simulink model "acc_mpc"  (R2021b)
settings: Solver=ode5  StartTime=0.0  StopTime=80  FixedStep=1/20  RelTol=1e-3
PreLoadFcn:
  | mbxruntime.callbacks.PreLoadFcn(bdroot);
PostLoadFcn:
  | mbxruntime.callbacks.PostLoadFcn(bdroot);
InitFcn:
  | mbxruntime.callbacks.InitFcn(bdroot);
StartFcn:
  | mbxruntime.callbacks.StartFcn(bdroot);
StopFcn:
  | mbxruntime.callbacks.StopFcn(bdroot);
model workspace: external: MAT-File .\kea_demo_0218_cs_hws.mat (data not in the file)
undefined symbols (not defined in the file): DiscIntNeverNeededParam, kea_demo_0218_cs_1d5c9b61e8e009e5, kea_demo_0218_cs_4669f259e7287783, kea_demo_0218_cs_87ee11d7829c0052, kea_demo_0218_cs_Audi_A3_1_Dynamics_Simple_initialPitch, kea_demo_0218_cs_Audi_A3_1_Dynamics_Simple_initialRoll, kea_demo_0218_cs_Audi_A3_1_Dynamics_Simple_initialX, kea_demo_0218_cs_Audi_A3_1_Dynamics_Simple_initialY, kea_demo_0218_cs_Audi_A3_1_Dynamics_Simple_initialYaw, kea_demo_0218_cs_Audi_A3_1_Dynamics_Simple_initialZ, kea_demo_0218_cs_Audi_A3_1_PathFollower_Preview_1_PathUniqueID, kea_demo_0218_cs_Roewe_550_S_Sedan_1_Dynamics_Simple_initialX, kea_demo_0218_cs_Roewe_550_S_Sedan_1_Dynamics_Simple_initialY, kea_demo_0218_cs_Roewe_550_S_Sedan_1_Dynamics_Simple_initialYaw, kea_demo_0218_cs_Roewe_550_S_Sedan_1_Dynamics_Simple_initialZ, mbxruntime, warningInitialVelocity, x0
libraries: simulink x56, simulink_extras x18, mpcadaslib x1
(part 2 of 8)

== system acc_mpc/Synchronizer ==
  Bus Selector1 : BusSelector  OutputSignals=FederateStopped
  Stop Simulation : Stop
  sfun_Synchronizer : S-Function  FunctionName=sfun_Synchronizer  Parameters=SampleTime  SFunctionDeploymentMode=off  EnableBusSupport=off  mask(Legacy Function){SFunctionSpec=void prescan_synchronizer_outputFcn(void ** work1, PRESCAN_SYNCHRONIZEDATA y1[1]), SampleTime=TimeStep, ShowSpec=on}
      mask prompts: SampleTime "Sample time (-1 for inherited):"; ShowSpec "Display function specification"
      mask help:
      | This block allows you to call the legacy functions specified by the following Legacy Code Tool definition:
      | def.SFunctionName = 'sfun_Synchronizer';
      | def.OutputFcnSpec = 'void prescan_synchronizer_outputFcn(void ** work1, PRESCAN_TIMESTAMPDATA u1[1], PRESCAN_SYNCHRONIZEDATA y1[1])';
      | def.StartFcnSpec = 'void prescan_synchronizer_startFcn(void ** work1)';
      | def.TerminateFcnSpec = 'void prescan_synchronizer_terminateFcn(void ** work1)';
      | def.HeaderFiles = {'prescan_synchronizer_data.h'};
      | def.HostLibFiles = {'sensorinterfaced.lib'};
      | def.IncPaths = {'src', 'C:\prescandev\vislibrary\vis\..\pimp\include\sensors\InterfaceRTW'};
      | def.SrcPaths = {'src'};
      | def.LibPaths = {'C:\\prescandev\\vislibrary_build\lib'};
      | def.SampleTime = 'parameterized';
      | def.Options.language = 'C';
      mask Help: <p>This block was generated automatically by the Legacy Code Tool. For detailed help on this tool, call<a href="matlab:legacy_code('help')"> legacy_code('help')</a>.</p>
      mask Callback ShowSpec:
      | if strcmp(get_param(gcbh, 'ShowSpec'), 'on')
      |   set_param(gcbh, 'MaskDisplay', sprintf('fprintf(''%s'');', get_param(gcbh, 'SFunctionSpec')));
      | else
      |   set_param(gcbh, 'MaskDisplay', sprintf('fprintf(''%s'');', get_param(gcbh, 'FunctionName')));
      | end
      mask Display: fprintf('void prescan_synchronizer_outputFcn(void ** work1, PRESCAN_SYNCHRONIZEDATA y1[1])');
  wires:
  sfun_Synchronizer/1 -> Bus Selector1/1
  Bus Selector1/1 -> Stop Simulation/1  "<FederateStopped>"

== system acc_mpc/Audi_A3_1/AIR_1_Demux ==
  AIR : Inport  OutDataTypeStr=Bus: PRESCAN_AIRSENSORMESSAGE
  Activate_Switch : Subsystem
      mask Display: text(5,10,'')
  Bus Selector : BusSelector  OutputSignals=DATA.Range,DATA.Azimuth,DATA.Elevation,DATA.ID,DATA.Velocity,DATA.Heading,HEADER.timestamp
  Data Type Conversion : DataTypeConversion  OutDataTypeStr=double
  For Iterator : ForIterator  ResetStates=reset  IterationLimit=detectableObjects
  Selector : Selector  InputPortWidth=detectableObjects  IndexOptions=Index vector (port)  Indices=[1 3]  OutputSizes=1
  Signal2ArrayOfSignals1 : Subsystem  mask{VECTORLENGTH=detectableObjects}
      mask prompts: VECTORLENGTH "Length of vector"
  Signal2ArrayOfSignals2 : Subsystem  mask{VECTORLENGTH=detectableObjects}
      mask prompts: VECTORLENGTH "Length of vector"
  Signal2ArrayOfSignals3 : Subsystem  mask{VECTORLENGTH=detectableObjects}
      mask prompts: VECTORLENGTH "Length of vector"
  Signal2ArrayOfSignals4 : Subsystem  mask{VECTORLENGTH=detectableObjects}
      mask prompts: VECTORLENGTH "Length of vector"
  Signal2ArrayOfSignals5 : Subsystem  mask{VECTORLENGTH=detectableObjects}
      mask prompts: VECTORLENGTH "Length of vector"
  Signal2ArrayOfSignals6 : Subsystem  mask{VECTORLENGTH=detectableObjects}
      mask prompts: VECTORLENGTH "Length of vector"
  Signal2ArrayOfSignals7 : Subsystem  mask{VECTORLENGTH=detectableObjects}
      mask prompts: VECTORLENGTH "Length of vector"
  Range [m] : Outport  VectorParamsAs1DForOutWhenUnconnected=off
  Azimuth [deg] : Outport  Port=2  VectorParamsAs1DForOutWhenUnconnected=off
  Elevation [deg] : Outport  Port=3  VectorParamsAs1DForOutWhenUnconnected=off
  ID [-] : Outport  Port=4  VectorParamsAs1DForOutWhenUnconnected=off
  Velocity [m/s] : Outport  Port=5  VectorParamsAs1DForOutWhenUnconnected=off
  Heading [deg] : Outport  Port=6  VectorParamsAs1DForOutWhenUnconnected=off
  Timestamp [s] : Outport  Port=7  VectorParamsAs1DForOutWhenUnconnected=off
  wires:
  Signal2ArrayOfSignals7/1(ArrayofElements) -> Timestamp [s]/1
  Bus Selector/7 -> Signal2ArrayOfSignals7/2(Element)  "<timestamp>"
  Activate_Switch/1(On/Off) -> Heading [deg]/1
  AIR/1 -> Selector/1
  For Iterator/1 -> Signal2ArrayOfSignals6/1(LoopIndex), Signal2ArrayOfSignals5/1(LoopIndex), Signal2ArrayOfSignals4/1(LoopIndex), Signal2ArrayOfSignals3/1(LoopIndex), Signal2ArrayOfSignals1/1(LoopIndex), Signal2ArrayOfSignals2/1(LoopIndex), Signal2ArrayOfSignals7/1(LoopIndex), Selector/2
  Selector/1 -> Bus Selector/1
  Bus Selector/1 -> Signal2ArrayOfSignals2/2(Element)  "<Range>"
  Signal2ArrayOfSignals2/1(ArrayofElements) -> Range [m]/1
  Signal2ArrayOfSignals1/1(ArrayofElements) -> Azimuth [deg]/1
  Bus Selector/2 -> Signal2ArrayOfSignals1/2(Element)  "<Azimuth>"
  Signal2ArrayOfSignals3/1(ArrayofElements) -> Elevation [deg]/1
  Bus Selector/3 -> Signal2ArrayOfSignals3/2(Element)  "<Elevation>"
  Signal2ArrayOfSignals4/1(ArrayofElements) -> Activate_Switch/1(BeamID), Data Type Conversion/1
  Bus Selector/4 -> Signal2ArrayOfSignals4/2(Element)  "<ID>"
  Signal2ArrayOfSignals5/1(ArrayofElements) -> Velocity [m/s]/1
  Bus Selector/5 -> Signal2ArrayOfSignals5/2(Element)  "<Velocity>"
  Signal2ArrayOfSignals6/1(ArrayofElements) -> Activate_Switch/2(Heading)
  Bus Selector/6 -> Signal2ArrayOfSignals6/2(Element)  "<Heading>"
  Data Type Conversion/1 -> ID [-]/1

== system acc_mpc/Audi_A3_1/AIR_3_Demux ==
  AIR : Inport  OutDataTypeStr=Bus: PRESCAN_AIRSENSORMESSAGE
  Activate_Switch : Subsystem
      mask Display: text(5,10,'')
  Bus Selector : BusSelector  OutputSignals=DATA.Range,DATA.Azimuth,DATA.Elevation,DATA.ID,DATA.Velocity,DATA.Heading,HEADER.timestamp
  Data Type Conversion : DataTypeConversion  OutDataTypeStr=double
  For Iterator : ForIterator  ResetStates=reset  IterationLimit=detectableObjects
  Selector : Selector  InputPortWidth=detectableObjects  IndexOptions=Index vector (port)  Indices=[1 3]  OutputSizes=1
  Signal2ArrayOfSignals1 : Subsystem  mask{VECTORLENGTH=detectableObjects}
      mask prompts: VECTORLENGTH "Length of vector"
  Signal2ArrayOfSignals2 : Subsystem  mask{VECTORLENGTH=detectableObjects}
      mask prompts: VECTORLENGTH "Length of vector"
  Signal2ArrayOfSignals3 : Subsystem  mask{VECTORLENGTH=detectableObjects}
      mask prompts: VECTORLENGTH "Length of vector"
  Signal2ArrayOfSignals4 : Subsystem  mask{VECTORLENGTH=detectableObjects}
      mask prompts: VECTORLENGTH "Length of vector"
  Signal2ArrayOfSignals5 : Subsystem  mask{VECTORLENGTH=detectableObjects}
      mask prompts: VECTORLENGTH "Length of vector"
  Signal2ArrayOfSignals6 : Subsystem  mask{VECTORLENGTH=detectableObjects}
      mask prompts: VECTORLENGTH "Length of vector"
  Signal2ArrayOfSignals7 : Subsystem  mask{VECTORLENGTH=detectableObjects}
      mask prompts: VECTORLENGTH "Length of vector"
  Range [m] : Outport  VectorParamsAs1DForOutWhenUnconnected=off
  Azimuth [deg] : Outport  Port=2  VectorParamsAs1DForOutWhenUnconnected=off
  Elevation [deg] : Outport  Port=3  VectorParamsAs1DForOutWhenUnconnected=off
  ID [-] : Outport  Port=4  VectorParamsAs1DForOutWhenUnconnected=off
  Velocity [m/s] : Outport  Port=5  VectorParamsAs1DForOutWhenUnconnected=off
  Heading [deg] : Outport  Port=6  VectorParamsAs1DForOutWhenUnconnected=off
  Timestamp [s] : Outport  Port=7  VectorParamsAs1DForOutWhenUnconnected=off
  wires:
  Signal2ArrayOfSignals7/1(ArrayofElements) -> Timestamp [s]/1
  Bus Selector/7 -> Signal2ArrayOfSignals7/2(Element)  "<timestamp>"
  Activate_Switch/1(On/Off) -> Heading [deg]/1
  AIR/1 -> Selector/1
  For Iterator/1 -> Signal2ArrayOfSignals6/1(LoopIndex), Signal2ArrayOfSignals5/1(LoopIndex), Signal2ArrayOfSignals4/1(LoopIndex), Signal2ArrayOfSignals3/1(LoopIndex), Signal2ArrayOfSignals1/1(LoopIndex), Signal2ArrayOfSignals2/1(LoopIndex), Signal2ArrayOfSignals7/1(LoopIndex), Selector/2
  Selector/1 -> Bus Selector/1
  Bus Selector/1 -> Signal2ArrayOfSignals2/2(Element)  "<Range>"
  Signal2ArrayOfSignals2/1(ArrayofElements) -> Range [m]/1
  Signal2ArrayOfSignals1/1(ArrayofElements) -> Azimuth [deg]/1
  Bus Selector/2 -> Signal2ArrayOfSignals1/2(Element)  "<Azimuth>"
  Signal2ArrayOfSignals3/1(ArrayofElements) -> Elevation [deg]/1
  Bus Selector/3 -> Signal2ArrayOfSignals3/2(Element)  "<Elevation>"
  Signal2ArrayOfSignals4/1(ArrayofElements) -> Activate_Switch/1(BeamID), Data Type Conversion/1
  Bus Selector/4 -> Signal2ArrayOfSignals4/2(Element)  "<ID>"
  Signal2ArrayOfSignals5/1(ArrayofElements) -> Velocity [m/s]/1
  Bus Selector/5 -> Signal2ArrayOfSignals5/2(Element)  "<Velocity>"
  Signal2ArrayOfSignals6/1(ArrayofElements) -> Activate_Switch/2(Heading)
  Bus Selector/6 -> Signal2ArrayOfSignals6/2(Element)  "<Heading>"
  Data Type Conversion/1 -> ID [-]/1

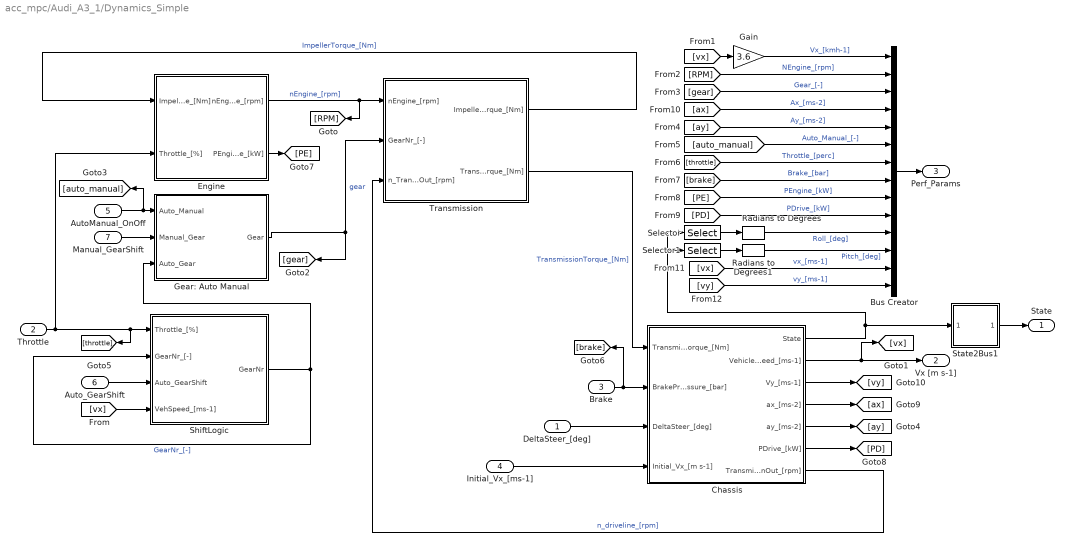
== system acc_mpc/Audi_A3_1/Dynamics_Simple ==
  DeltaSteer_[deg] : Inport
  Throttle : Inport  Port=2
  Brake : Inport  Port=3
  Initial_Vx_[ms-1] : Inport  Port=4
  AutoManual_OnOff : Inport  Port=5
  Auto_GearShift : Inport  Port=6
  Manual_GearShift : Inport  Port=7
  Bus Creator : BusCreator  Inputs=14
  Chassis : Subsystem
      mask Display: image(imread('Chassis.png'));
  Engine : Subsystem
      mask Display: image(imread('Engine.png'));
  Gain : Gain  Gain=3.6
  Gear: Auto Manual : Subsystem
  Radians to Degrees : simulink_extras/Transformations/Radians to Degrees
  Radians to Degrees1 : simulink_extras/Transformations/Radians to Degrees
  Selector : Selector  InputPortWidth=9  IndexOptions=Index vector (dialog)  Indices=7  OutputSizes=1
  Selector1 : Selector  InputPortWidth=9  IndexOptions=Index vector (dialog)  Indices=8  OutputSizes=1
  ShiftLogic : Subsystem
      mask Display: image(imread('Gearshift.png'));
  State2Bus1 : Subsystem  Tag=State  Priority=0  LoadFcn=load PrescanStateActuatorData  mask(PreScan Sink Block: State){x0=initialX, y0=initialY, z0=initialZ, Roll0=initialRoll, Pitch0=initialPitch, Yaw0=initialYaw, TimeStep=TimeStep}
      mask prompts: x0 "Ini x-position VEHICLE wrt GLOBAL axis system [m]"; y0 "Ini y-position VEHICLE wrt GLOBAL axis system [m]"; z0 "Ini z-position VEHICLE wrt GLOBAL axis system [m]"; Roll0 "Ini roll-angle BODY wrt VEHICLE axis system [deg]"; Pitch0 "Ini pitch-angle BODY wrt VEHICLE axis system [deg]"; Yaw0 "Ini yaw-angle VEHICLE wrt GLOBAL axis system [deg]"; TimeStep "Auto-Assigned: Upload Period [s]"
      mask help:
      | The Actor State contains a vector signal of size (9x1), containing the following signals:
      |
      | -  Position                  (x,y,z)                                     [m]
      | -  Velocity                  (vx,vy,vz)                               [m/s]
      | -  Angles                    (Roll, Pitch, Yaw)                   [rad]
      |
      | The Actor state is defined in the global axis system.
      | The state is superponed on the Initial position defined in the GUI.
      |
      | For more information, please click Help.
      settings: DeleteFcn=PreScanBlockDeleteFcn;
      mask Help: eval('openHelp(222)')
      mask Display: image(imread('State.png'))
  Transmission : Subsystem
      mask Display: image(imread('Transmission.png'));
  State : Outport  VectorParamsAs1DForOutWhenUnconnected=off
  Vx [m s-1] : Outport  Port=2  VectorParamsAs1DForOutWhenUnconnected=off
  Perf_Params : Outport  Port=3  VectorParamsAs1DForOutWhenUnconnected=off
  wires:
  State2Bus1/1(StateBus) -> State/1
  [vy] -> Bus Creator/14  "vy_[ms-1]"
  [vx] -> Bus Creator/13  "vx_[ms-1]"
  Chassis/7(TransmissionOut_[rpm]) -> Transmission/3(n_TransmissionOut_[rpm])  "n_driveline_[rpm]"
  Chassis/6(PDrive_[kW]) -> [PD]
  Chassis/5(ay_[ms-2]) -> [ay]
  Chassis/4(ax_[ms-2]) -> [ax]
  Chassis/3(Vy_[ms-1]) -> [vy]
  [vx] -> ShiftLogic/4(VehSpeed_[ms-1])
  Gear: Auto Manual/1(Gear) -> Transmission/2(GearNr_[-]), [gear]  "gear"
  Manual_GearShift/1 -> Gear: Auto Manual/2(Manual_Gear)
  AutoManual_OnOff/1 -> Gear: Auto Manual/1(Auto_Manual), [auto_manual]
  Chassis/2(VehicleSpeed_[ms-1]) -> [vx], Vx [m s-1]/1
  Auto_GearShift/1 -> ShiftLogic/3(Auto_GearShift)
  Throttle/1 -> Engine/2(Throttle_[%]), ShiftLogic/1(Throttle_[%]), [throttle]
  Initial_Vx_[ms-1]/1 -> Chassis/4(Initial_Vx_[m s-1])
  DeltaSteer_[deg]/1 -> Chassis/3(DeltaSteer_[deg])
  Chassis/1(State) -> Selector/1, Selector1/1, State2Bus1/1(State)
  Brake/1 -> [brake], Chassis/2(BrakePressure_[bar])
  Engine/1(nEngine_[rpm]) -> [RPM], Transmission/1(nEngine_[rpm])  "nEngine_[rpm]"
  ShiftLogic/1(GearNr) -> Gear: Auto Manual/3(Auto_Gear), ShiftLogic/2(GearNr_[-])  "GearNr_[-]"
  Transmission/2(TransmissionTorque_[Nm]) -> Chassis/1(TransmissionTorque_[Nm])  "TransmissionTorque_[Nm]"
  Transmission/1(ImpellerTorque_[Nm]) -> Engine/1(ImpellerTorque_[Nm])  "ImpellerTorque_[Nm]"
  Gain/1 -> Bus Creator/1  "Vx_[kmh-1]"
  [RPM] -> Bus Creator/2  "NEngine_[rpm]"
  [gear] -> Bus Creator/3  "Gear_[-]"
  [ay] -> Bus Creator/5  "Ay_[ms-2]"
  [auto_manual] -> Bus Creator/6  "Auto_Manual_[-]"
  [throttle] -> Bus Creator/7  "Throttle_[perc]"
  [brake] -> Bus Creator/8  "Brake_[bar]"
  Engine/2(PEngine_[kW]) -> [PE]
  Bus Creator/1 -> Perf_Params/1
  [PE] -> Bus Creator/9  "PEngine_[kW]"
  Radians to Degrees/1 -> Bus Creator/11  "Roll_[deg]"
  Radians to Degrees1/1 -> Bus Creator/12  "Pitch_[deg]"
  [PD] -> Bus Creator/10  "PDrive_[kW]"
  Selector/1 -> Radians to Degrees/1
  Selector1/1 -> Radians to Degrees1/1
  [vx] -> Gain/1
  [ax] -> Bus Creator/4  "Ax_[ms-2]"

== system acc_mpc/Audi_A3_1/PathFollower_Preview_1 ==
  ActorOffset_Left(+) / Right(-) [m] : Inport
  position x,y,Y [m,m,deg] : Inport  Port=2
  Initial Velocity [m/s] : Inport  Port=3
  Desired Velocity [m/s] : Inport  Port=4
  velocity [m/s] : Inport  Port=5
  vx [m/s] : Inport  Port=6
  vy [m/s] : Inport  Port=7
  Yaw rate [deg/s] : Inport  Port=8
  CorneringStiffness_Tyres_Front [N/rad] : Inport  Port=9
  CorneringStiffness_Tyres_Rear [N/rad] : Inport  Port=10
  steering_ratio[-] : Inport  Port=11
  LateralController : Subsystem
  LongitudinalController : Subsystem
  delta_steerwheel [deg] : Outport  VectorParamsAs1DForOutWhenUnconnected=off
  throttle [%] : Outport  Port=2  VectorParamsAs1DForOutWhenUnconnected=off
  brake pressure [bar] : Outport  Port=3  VectorParamsAs1DForOutWhenUnconnected=off
  v0 [m/s] : Outport  Port=4  VectorParamsAs1DForOutWhenUnconnected=off
  Auto_GearShift : Outport  Port=5  VectorParamsAs1DForOutWhenUnconnected=off
  Actor/Traj_distance [m] : Outport  Port=6  VectorParamsAs1DForOutWhenUnconnected=off
  Actor/Traj_angle [deg] : Outport  Port=7  VectorParamsAs1DForOutWhenUnconnected=off
  wires:
  LateralController/3(delta_steerwheel [deg]) -> delta_steerwheel [deg]/1
  steering_ratio[-]/1 -> LateralController/8(steering_ratio[-])
  CorneringStiffness_Tyres_Rear [N/rad]/1 -> LateralController/7(CorneringStiffness_Tyres_Rear [N/rad])
  CorneringStiffness_Tyres_Front [N/rad]/1 -> LateralController/6(CorneringStiffness_Tyres_Front [N/rad])
  Yaw rate [deg/s]/1 -> LateralController/5(Yaw rate [deg/s])
  vy [m/s]/1 -> LateralController/4(vy [m/s])
  vx [m/s]/1 -> LateralController/3(vx [m/s])
  position x,y,Y [m,m,deg]/1 -> LateralController/2(position x,y,Y [m,m,deg])
  ActorOffset_Left(+) / Right(-) [m]/1 -> LateralController/1(ActorOffset_Left(+) / Right(-) [m])
  LateralController/2(Actor/Traj_angle [deg]) -> Actor/Traj_angle [deg]/1
  LateralController/1(Actor/Traj_distance [m]) -> Actor/Traj_distance [m]/1
  velocity [m/s]/1 -> LongitudinalController/1(v_actual [m/s])
  LongitudinalController/1(throttle [%]) -> throttle [%]/1
  Desired Velocity [m/s]/1 -> LongitudinalController/2(Desired Velocity [m/s])
  Initial Velocity [m/s]/1 -> LongitudinalController/3(Initial Velocity [m/s])
  LongitudinalController/2(brake pressure [bar]) -> brake pressure [bar]/1
  LongitudinalController/3(v0 [m/s]) -> v0 [m/s]/1
  LongitudinalController/4(Auto_GearShift) -> Auto_GearShift/1

== system acc_mpc/Audi_A3_1/SELF_Demux ==
  SELF : Inport  OutDataTypeStr=Bus: PRESCAN_SELFSENSORDATA
  Bus Selector : BusSelector  OutputSignals=PositionX,PositionY,PositionZ,OrientationRoll,OrientationPitch,OrientationYaw,Velocity,Yaw_rate,Lat,Long,Alt,TimeStamp
  Demux2 : Demux  Outputs=3
  Gain : Gain  Gain=180/pi
  Gain1 : Gain  Gain=180/pi
  Vector Concatenate1 : Concatenate  NumInputs=3
  compas converter : Subsystem
  x [m] : Outport  VectorParamsAs1DForOutWhenUnconnected=off
  y [m] : Outport  Port=2  VectorParamsAs1DForOutWhenUnconnected=off
  z [m] : Outport  Port=3  VectorParamsAs1DForOutWhenUnconnected=off
  rotx [deg] : Outport  Port=4  VectorParamsAs1DForOutWhenUnconnected=off
  roty [deg] : Outport  Port=5  VectorParamsAs1DForOutWhenUnconnected=off
  rotz [deg] : Outport  Port=6  VectorParamsAs1DForOutWhenUnconnected=off
  GPS lat [deg] : Outport  Port=7  VectorParamsAs1DForOutWhenUnconnected=off
  GPS long [deg] : Outport  Port=8  VectorParamsAs1DForOutWhenUnconnected=off
  GPS alt [m] : Outport  Port=9  VectorParamsAs1DForOutWhenUnconnected=off
  velocity [m/s] : Outport  Port=10  VectorParamsAs1DForOutWhenUnconnected=off
  heading [deg] : Outport  Port=11  VectorParamsAs1DForOutWhenUnconnected=off
  yaw rate [deg/s] : Outport  Port=12  VectorParamsAs1DForOutWhenUnconnected=off
  TimeStamp [s] : Outport  Port=13  VectorParamsAs1DForOutWhenUnconnected=off
  wires:
  Bus Selector/12 -> TimeStamp [s]/1  "<TimeStamp>"
  Bus Selector/11 -> GPS alt [m]/1  "<Alt>"
  Bus Selector/10 -> GPS long [deg]/1  "<Long>"
  Bus Selector/9 -> GPS lat [deg]/1  "<Lat>"
  Bus Selector/8 -> Gain1/1  "<Yaw_rate>"
  Bus Selector/7 -> velocity [m/s]/1  "<Velocity>"
  Bus Selector/6 -> compas converter/1(rotz [rad]), Vector Concatenate1/3  "<OrientationYaw>"
  Bus Selector/5 -> Vector Concatenate1/2  "<OrientationPitch>"
  Bus Selector/4 -> Vector Concatenate1/1  "<OrientationRoll>"
  Vector Concatenate1/1 -> Gain/1
  Bus Selector/3 -> z [m]/1  "<PositionZ>"
  Bus Selector/2 -> y [m]/1  "<PositionY>"
  Bus Selector/1 -> x [m]/1  "<PositionX>"
  SELF/1 -> Bus Selector/1
  Gain/1 -> Demux2/1
  Demux2/1 -> rotx [deg]/1
  Demux2/2 -> roty [deg]/1
  Demux2/3 -> rotz [deg]/1
  compas converter/1(heading [deg]) -> heading [deg]/1
  Gain1/1 -> yaw rate [deg/s]/1

== system acc_mpc/Audi_A3_1/Speed ==
  BusSelector : BusSelector  OutputSignals=value
  sfun : S-Function  LoadFcn=load('PrescanScalarData.mat')  FunctionName=sfun_ProtobufScalarReader  Parameters=mbxruntime.parameters.convert(model), mbxruntime.parameters.convert(path), mbxruntime.parameters.convert(myType), mbxruntime.parameters.convert(timestep)  SFunctionDeploymentMode=off  EnableBusSupport=off  mask(PreScan Source Block: Protobuffer Scalar Reader){model=uint8(['pimp/scenariomodel' 0]), path=uint8(['catalogs/maneuverCatalog/maneuver:1/event:0/startConditions:0/condition:1/byEntity/speed/value' 0]), myType=uint8(['double' 0]), timestep=0}
      mask prompts: model "Data Model:"; path "Data Model Path:"; myType "Data Type:"; timestep "MATLAB timestep:"
      mask help:
      | This block reads a scalar value from the pb file.
      |
      | The supported data types are:
      | - double
      | - single
      | - uint32
      | - int32
      mask Display: fprintf('sfun')
  Speed : Outport
  wires:
  sfun/1 -> BusSelector/1
  BusSelector/1 -> Speed/1  "<value>"

== system acc_mpc/Audi_A3_1/State2PathFollowerCnv ==
  State BUS : Inport  OutDataTypeStr=Bus: PRESCAN_STATEACTUATORDATA
  Bus Selector : BusSelector  OutputSignals=AngularVelocityYaw,VelocityX,VelocityY,PositionX,PositionY,OrientationYaw
  Radians to Degrees : simulink_extras/Transformations/Radians to Degrees
  Radians to Degrees1 : simulink_extras/Transformations/Radians to Degrees
  SELF2PathFollowerMux : Mux  Tag=SELF2PathFollowerMux  Inputs=3
  velocity magnitude : Math  Operator=hypot  SignedPower=on  SaturateOnIntegerOverflow=on
  Yaw rate [deg/s] : Outport  VectorParamsAs1DForOutWhenUnconnected=off
  velocity [m/s] : Outport  Port=2  VectorParamsAs1DForOutWhenUnconnected=off
  position x,y,Y [m,m,deg] : Outport  Port=3  VectorParamsAs1DForOutWhenUnconnected=off
  wires:
  Radians to Degrees1/1 -> Yaw rate [deg/s]/1
  Bus Selector/1 -> Radians to Degrees1/1  "<AngularVelocityYaw>"
  velocity magnitude/1 -> velocity [m/s]/1
  SELF2PathFollowerMux/1 -> position x,y,Y [m,m,deg]/1
  State BUS/1 -> Bus Selector/1
  Bus Selector/2 -> velocity magnitude/1  "<VelocityX>"
  Bus Selector/3 -> velocity magnitude/2  "<VelocityY>"
  Radians to Degrees/1 -> SELF2PathFollowerMux/3
  Bus Selector/6 -> Radians to Degrees/1  "<OrientationYaw>"
  Bus Selector/4 -> SELF2PathFollowerMux/1  "<PositionX>"
  Bus Selector/5 -> SELF2PathFollowerMux/2  "<PositionY>"

== system acc_mpc/Audi_A3_1/Subsystem ==
  Acceleration : Inport
  Lead Val : Inport  Port=2
  If Action Subsystem : Subsystem  TreatAsAtomicUnit=on
  If Action Subsystem2 : Subsystem  TreatAsAtomicUnit=on
  If1 : If  IfExpression=u1==0
  Merge : Merge
  Merge1 : Merge
  Throttle : Outport
  Brake : Outport  Port=2
  wires:
  Lead Val/1 -> If1/1
  If1/2 -> If Action Subsystem2/Action
  Acceleration/1 -> If Action Subsystem2/1(Acceleration)
  If Action Subsystem2/1(Throttle) -> Merge/1
  If Action Subsystem2/2(Brake) -> Merge1/1
  Merge/1 -> Throttle/1
  If1/1 -> If Action Subsystem/Action
  If Action Subsystem/1(Throttle) -> Merge/2
  If Action Subsystem/2(Brake) -> Merge1/2
  Merge1/1 -> Brake/1

== system acc_mpc/Roewe_550_S_Sedan_1/AIR_2_Demux ==
  AIR : Inport  OutDataTypeStr=Bus: PRESCAN_AIRSENSORMESSAGE
  Activate_Switch : Subsystem
      mask Display: text(5,10,'')
  Bus Selector : BusSelector  OutputSignals=DATA.Range,DATA.Azimuth,DATA.Elevation,DATA.ID,DATA.Velocity,DATA.Heading,HEADER.timestamp
  Data Type Conversion : DataTypeConversion  OutDataTypeStr=double
  For Iterator : ForIterator  ResetStates=reset  IterationLimit=detectableObjects
  Selector : Selector  InputPortWidth=detectableObjects  IndexOptions=Index vector (port)  Indices=[1 3]  OutputSizes=1
  Signal2ArrayOfSignals1 : Subsystem  mask{VECTORLENGTH=detectableObjects}
      mask prompts: VECTORLENGTH "Length of vector"
  Signal2ArrayOfSignals2 : Subsystem  mask{VECTORLENGTH=detectableObjects}
      mask prompts: VECTORLENGTH "Length of vector"
  Signal2ArrayOfSignals3 : Subsystem  mask{VECTORLENGTH=detectableObjects}
      mask prompts: VECTORLENGTH "Length of vector"
  Signal2ArrayOfSignals4 : Subsystem  mask{VECTORLENGTH=detectableObjects}
      mask prompts: VECTORLENGTH "Length of vector"
  Signal2ArrayOfSignals5 : Subsystem  mask{VECTORLENGTH=detectableObjects}
      mask prompts: VECTORLENGTH "Length of vector"
  Signal2ArrayOfSignals6 : Subsystem  mask{VECTORLENGTH=detectableObjects}
      mask prompts: VECTORLENGTH "Length of vector"
  Signal2ArrayOfSignals7 : Subsystem  mask{VECTORLENGTH=detectableObjects}
      mask prompts: VECTORLENGTH "Length of vector"
  Range [m] : Outport  VectorParamsAs1DForOutWhenUnconnected=off
  Azimuth [deg] : Outport  Port=2  VectorParamsAs1DForOutWhenUnconnected=off
  Elevation [deg] : Outport  Port=3  VectorParamsAs1DForOutWhenUnconnected=off
  ID [-] : Outport  Port=4  VectorParamsAs1DForOutWhenUnconnected=off
  Velocity [m/s] : Outport  Port=5  VectorParamsAs1DForOutWhenUnconnected=off
  Heading [deg] : Outport  Port=6  VectorParamsAs1DForOutWhenUnconnected=off
  Timestamp [s] : Outport  Port=7  VectorParamsAs1DForOutWhenUnconnected=off
  wires:
  Signal2ArrayOfSignals7/1(ArrayofElements) -> Timestamp [s]/1
  Bus Selector/7 -> Signal2ArrayOfSignals7/2(Element)  "<timestamp>"
  Activate_Switch/1(On/Off) -> Heading [deg]/1
  AIR/1 -> Selector/1
  For Iterator/1 -> Signal2ArrayOfSignals6/1(LoopIndex), Signal2ArrayOfSignals5/1(LoopIndex), Signal2ArrayOfSignals4/1(LoopIndex), Signal2ArrayOfSignals3/1(LoopIndex), Signal2ArrayOfSignals1/1(LoopIndex), Signal2ArrayOfSignals2/1(LoopIndex), Signal2ArrayOfSignals7/1(LoopIndex), Selector/2
  Selector/1 -> Bus Selector/1
  Bus Selector/1 -> Signal2ArrayOfSignals2/2(Element)  "<Range>"
  Signal2ArrayOfSignals2/1(ArrayofElements) -> Range [m]/1
  Signal2ArrayOfSignals1/1(ArrayofElements) -> Azimuth [deg]/1
  Bus Selector/2 -> Signal2ArrayOfSignals1/2(Element)  "<Azimuth>"
  Signal2ArrayOfSignals3/1(ArrayofElements) -> Elevation [deg]/1
  Bus Selector/3 -> Signal2ArrayOfSignals3/2(Element)  "<Elevation>"
  Signal2ArrayOfSignals4/1(ArrayofElements) -> Activate_Switch/1(BeamID), Data Type Conversion/1
  Bus Selector/4 -> Signal2ArrayOfSignals4/2(Element)  "<ID>"
  Signal2ArrayOfSignals5/1(ArrayofElements) -> Velocity [m/s]/1
  Bus Selector/5 -> Signal2ArrayOfSignals5/2(Element)  "<Velocity>"
  Signal2ArrayOfSignals6/1(ArrayofElements) -> Activate_Switch/2(Heading)
  Bus Selector/6 -> Signal2ArrayOfSignals6/2(Element)  "<Heading>"
  Data Type Conversion/1 -> ID [-]/1

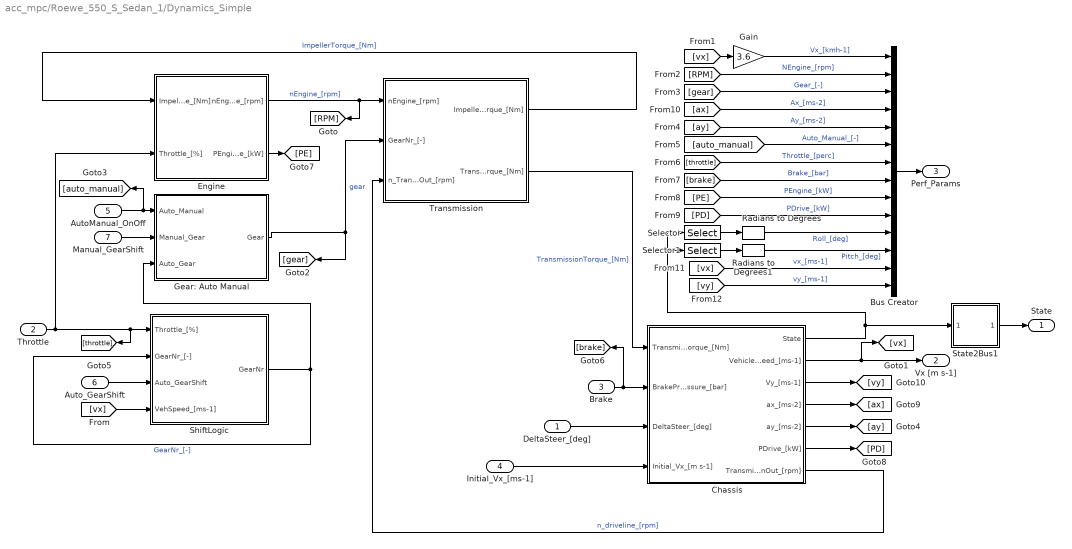
== system acc_mpc/Roewe_550_S_Sedan_1/Dynamics_Simple ==
  DeltaSteer_[deg] : Inport
  Throttle : Inport  Port=2
  Brake : Inport  Port=3
  Initial_Vx_[ms-1] : Inport  Port=4
  AutoManual_OnOff : Inport  Port=5
  Auto_GearShift : Inport  Port=6
  Manual_GearShift : Inport  Port=7
  Bus Creator : BusCreator  Inputs=14
  Chassis : Subsystem
      mask Display: image(imread('Chassis.png'));
  Engine : Subsystem
      mask Display: image(imread('Engine.png'));
  Gain : Gain  Gain=3.6
  Gear: Auto Manual : Subsystem
  Radians to Degrees : simulink_extras/Transformations/Radians to Degrees
  Radians to Degrees1 : simulink_extras/Transformations/Radians to Degrees
  Selector : Selector  InputPortWidth=9  IndexOptions=Index vector (dialog)  Indices=7  OutputSizes=1
  Selector1 : Selector  InputPortWidth=9  IndexOptions=Index vector (dialog)  Indices=8  OutputSizes=1
  ShiftLogic : Subsystem
      mask Display: image(imread('Gearshift.png'));
  State2Bus1 : Subsystem  Tag=State  Priority=0  LoadFcn=load PrescanStateActuatorData  mask(PreScan Sink Block: State){x0=initialX, y0=initialY, z0=initialZ, Roll0=initialRoll, Pitch0=initialPitch, Yaw0=initialYaw, TimeStep=TimeStep}
      mask prompts: x0 "Ini x-position VEHICLE wrt GLOBAL axis system [m]"; y0 "Ini y-position VEHICLE wrt GLOBAL axis system [m]"; z0 "Ini z-position VEHICLE wrt GLOBAL axis system [m]"; Roll0 "Ini roll-angle BODY wrt VEHICLE axis system [deg]"; Pitch0 "Ini pitch-angle BODY wrt VEHICLE axis system [deg]"; Yaw0 "Ini yaw-angle VEHICLE wrt GLOBAL axis system [deg]"; TimeStep "Auto-Assigned: Upload Period [s]"
      mask help:
      | The Actor State contains a vector signal of size (9x1), containing the following signals:
      |
      | -  Position                  (x,y,z)                                     [m]
      | -  Velocity                  (vx,vy,vz)                               [m/s]
      | -  Angles                    (Roll, Pitch, Yaw)                   [rad]
      |
      | The Actor state is defined in the global axis system.
      | The state is superponed on the Initial position defined in the GUI.
      |
      | For more information, please click Help.
      settings: DeleteFcn=PreScanBlockDeleteFcn;
      mask Help: eval('openHelp(222)')
      mask Display: image(imread('State.png'))
  Transmission : Subsystem
      mask Display: image(imread('Transmission.png'));
  State : Outport  VectorParamsAs1DForOutWhenUnconnected=off
  Vx [m s-1] : Outport  Port=2  VectorParamsAs1DForOutWhenUnconnected=off
  Perf_Params : Outport  Port=3  VectorParamsAs1DForOutWhenUnconnected=off
  wires:
  State2Bus1/1(StateBus) -> State/1
  [vy] -> Bus Creator/14  "vy_[ms-1]"
  [vx] -> Bus Creator/13  "vx_[ms-1]"
  Chassis/7(TransmissionOut_[rpm]) -> Transmission/3(n_TransmissionOut_[rpm])  "n_driveline_[rpm]"
  Chassis/6(PDrive_[kW]) -> [PD]
  Chassis/5(ay_[ms-2]) -> [ay]
  Chassis/4(ax_[ms-2]) -> [ax]
  Chassis/3(Vy_[ms-1]) -> [vy]
  [vx] -> ShiftLogic/4(VehSpeed_[ms-1])
  Gear: Auto Manual/1(Gear) -> Transmission/2(GearNr_[-]), [gear]  "gear"
  Manual_GearShift/1 -> Gear: Auto Manual/2(Manual_Gear)
  AutoManual_OnOff/1 -> Gear: Auto Manual/1(Auto_Manual), [auto_manual]
  Chassis/2(VehicleSpeed_[ms-1]) -> [vx], Vx [m s-1]/1
  Auto_GearShift/1 -> ShiftLogic/3(Auto_GearShift)
  Throttle/1 -> Engine/2(Throttle_[%]), ShiftLogic/1(Throttle_[%]), [throttle]
  Initial_Vx_[ms-1]/1 -> Chassis/4(Initial_Vx_[m s-1])
  DeltaSteer_[deg]/1 -> Chassis/3(DeltaSteer_[deg])
  Chassis/1(State) -> Selector/1, Selector1/1, State2Bus1/1(State)
  Brake/1 -> [brake], Chassis/2(BrakePressure_[bar])
  Engine/1(nEngine_[rpm]) -> [RPM], Transmission/1(nEngine_[rpm])  "nEngine_[rpm]"
  ShiftLogic/1(GearNr) -> Gear: Auto Manual/3(Auto_Gear), ShiftLogic/2(GearNr_[-])  "GearNr_[-]"
  Transmission/2(TransmissionTorque_[Nm]) -> Chassis/1(TransmissionTorque_[Nm])  "TransmissionTorque_[Nm]"
  Transmission/1(ImpellerTorque_[Nm]) -> Engine/1(ImpellerTorque_[Nm])  "ImpellerTorque_[Nm]"
  Gain/1 -> Bus Creator/1  "Vx_[kmh-1]"
  [RPM] -> Bus Creator/2  "NEngine_[rpm]"
  [gear] -> Bus Creator/3  "Gear_[-]"
  [ay] -> Bus Creator/5  "Ay_[ms-2]"
  [auto_manual] -> Bus Creator/6  "Auto_Manual_[-]"
  [throttle] -> Bus Creator/7  "Throttle_[perc]"
  [brake] -> Bus Creator/8  "Brake_[bar]"
  Engine/2(PEngine_[kW]) -> [PE]
  Bus Creator/1 -> Perf_Params/1
  [PE] -> Bus Creator/9  "PEngine_[kW]"
  Radians to Degrees/1 -> Bus Creator/11  "Roll_[deg]"
  Radians to Degrees1/1 -> Bus Creator/12  "Pitch_[deg]"
  [PD] -> Bus Creator/10  "PDrive_[kW]"
  Selector/1 -> Radians to Degrees/1
  Selector1/1 -> Radians to Degrees1/1
  [vx] -> Gain/1
  [ax] -> Bus Creator/4  "Ax_[ms-2]"

== system acc_mpc/Roewe_550_S_Sedan_1/PathFollower_Preview_1 ==
  ActorOffset_Left(+) / Right(-) [m] : Inport
  position x,y,Y [m,m,deg] : Inport  Port=2
  Initial Velocity [m/s] : Inport  Port=3
  Desired Velocity [m/s] : Inport  Port=4
  velocity [m/s] : Inport  Port=5
  vx [m/s] : Inport  Port=6
  vy [m/s] : Inport  Port=7
  Yaw rate [deg/s] : Inport  Port=8
  CorneringStiffness_Tyres_Front [N/rad] : Inport  Port=9
  CorneringStiffness_Tyres_Rear [N/rad] : Inport  Port=10
  steering_ratio[-] : Inport  Port=11
  LateralController : Subsystem
  LongitudinalController : Subsystem
  delta_steerwheel [deg] : Outport  VectorParamsAs1DForOutWhenUnconnected=off
  throttle [%] : Outport  Port=2  VectorParamsAs1DForOutWhenUnconnected=off
  brake pressure [bar] : Outport  Port=3  VectorParamsAs1DForOutWhenUnconnected=off
  v0 [m/s] : Outport  Port=4  VectorParamsAs1DForOutWhenUnconnected=off
  Auto_GearShift : Outport  Port=5  VectorParamsAs1DForOutWhenUnconnected=off
  Actor/Traj_distance [m] : Outport  Port=6  VectorParamsAs1DForOutWhenUnconnected=off
  Actor/Traj_angle [deg] : Outport  Port=7  VectorParamsAs1DForOutWhenUnconnected=off
  wires:
  LateralController/3(delta_steerwheel [deg]) -> delta_steerwheel [deg]/1
  steering_ratio[-]/1 -> LateralController/8(steering_ratio[-])
  CorneringStiffness_Tyres_Rear [N/rad]/1 -> LateralController/7(CorneringStiffness_Tyres_Rear [N/rad])
  CorneringStiffness_Tyres_Front [N/rad]/1 -> LateralController/6(CorneringStiffness_Tyres_Front [N/rad])
  Yaw rate [deg/s]/1 -> LateralController/5(Yaw rate [deg/s])
  vy [m/s]/1 -> LateralController/4(vy [m/s])
  vx [m/s]/1 -> LateralController/3(vx [m/s])
  position x,y,Y [m,m,deg]/1 -> LateralController/2(position x,y,Y [m,m,deg])
  ActorOffset_Left(+) / Right(-) [m]/1 -> LateralController/1(ActorOffset_Left(+) / Right(-) [m])
  LateralController/2(Actor/Traj_angle [deg]) -> Actor/Traj_angle [deg]/1
  LateralController/1(Actor/Traj_distance [m]) -> Actor/Traj_distance [m]/1
  velocity [m/s]/1 -> LongitudinalController/1(v_actual [m/s])
  LongitudinalController/1(throttle [%]) -> throttle [%]/1
  Desired Velocity [m/s]/1 -> LongitudinalController/2(Desired Velocity [m/s])
  Initial Velocity [m/s]/1 -> LongitudinalController/3(Initial Velocity [m/s])
  LongitudinalController/2(brake pressure [bar]) -> brake pressure [bar]/1
  LongitudinalController/3(v0 [m/s]) -> v0 [m/s]/1
  LongitudinalController/4(Auto_GearShift) -> Auto_GearShift/1

== system acc_mpc/Roewe_550_S_Sedan_1/SELF_Demux ==
  SELF : Inport  OutDataTypeStr=Bus: PRESCAN_SELFSENSORDATA
  Bus Selector : BusSelector  OutputSignals=PositionX,PositionY,PositionZ,OrientationRoll,OrientationPitch,OrientationYaw,Velocity,Yaw_rate,Lat,Long,Alt,TimeStamp
  Demux2 : Demux  Outputs=3
  Gain : Gain  Gain=180/pi
  Gain1 : Gain  Gain=180/pi
  Vector Concatenate1 : Concatenate  NumInputs=3
  compas converter : Subsystem
  x [m] : Outport  VectorParamsAs1DForOutWhenUnconnected=off
  y [m] : Outport  Port=2  VectorParamsAs1DForOutWhenUnconnected=off
  z [m] : Outport  Port=3  VectorParamsAs1DForOutWhenUnconnected=off
  rotx [deg] : Outport  Port=4  VectorParamsAs1DForOutWhenUnconnected=off
  roty [deg] : Outport  Port=5  VectorParamsAs1DForOutWhenUnconnected=off
  rotz [deg] : Outport  Port=6  VectorParamsAs1DForOutWhenUnconnected=off
  GPS lat [deg] : Outport  Port=7  VectorParamsAs1DForOutWhenUnconnected=off
  GPS long [deg] : Outport  Port=8  VectorParamsAs1DForOutWhenUnconnected=off
  GPS alt [m] : Outport  Port=9  VectorParamsAs1DForOutWhenUnconnected=off
  velocity [m/s] : Outport  Port=10  VectorParamsAs1DForOutWhenUnconnected=off
  heading [deg] : Outport  Port=11  VectorParamsAs1DForOutWhenUnconnected=off
  yaw rate [deg/s] : Outport  Port=12  VectorParamsAs1DForOutWhenUnconnected=off
  TimeStamp [s] : Outport  Port=13  VectorParamsAs1DForOutWhenUnconnected=off
  wires:
  Bus Selector/12 -> TimeStamp [s]/1  "<TimeStamp>"
  Bus Selector/11 -> GPS alt [m]/1  "<Alt>"
  Bus Selector/10 -> GPS long [deg]/1  "<Long>"
  Bus Selector/9 -> GPS lat [deg]/1  "<Lat>"
  Bus Selector/8 -> Gain1/1  "<Yaw_rate>"
  Bus Selector/7 -> velocity [m/s]/1  "<Velocity>"
  Bus Selector/6 -> compas converter/1(rotz [rad]), Vector Concatenate1/3  "<OrientationYaw>"
  Bus Selector/5 -> Vector Concatenate1/2  "<OrientationPitch>"
  Bus Selector/4 -> Vector Concatenate1/1  "<OrientationRoll>"
  Vector Concatenate1/1 -> Gain/1
  Bus Selector/3 -> z [m]/1  "<PositionZ>"
  Bus Selector/2 -> y [m]/1  "<PositionY>"
  Bus Selector/1 -> x [m]/1  "<PositionX>"
  SELF/1 -> Bus Selector/1
  Gain/1 -> Demux2/1
  Demux2/1 -> rotx [deg]/1
  Demux2/2 -> roty [deg]/1
  Demux2/3 -> rotz [deg]/1
  compas converter/1(heading [deg]) -> heading [deg]/1
  Gain1/1 -> yaw rate [deg/s]/1

== system acc_mpc/Roewe_550_S_Sedan_1/Speed ==
  BusSelector : BusSelector  OutputSignals=value
  sfun : S-Function  LoadFcn=load('PrescanScalarData.mat')  FunctionName=sfun_ProtobufScalarReader  Parameters=mbxruntime.parameters.convert(model), mbxruntime.parameters.convert(path), mbxruntime.parameters.convert(myType), mbxruntime.parameters.convert(timestep)  SFunctionDeploymentMode=off  EnableBusSupport=off  mask(PreScan Source Block: Protobuffer Scalar Reader){model=uint8(['pimp/scenariomodel' 0]), path=uint8(['catalogs/maneuverCatalog/maneuver:0/event:0/startConditions:0/condition:1/byEntity/speed/value' 0]), myType=uint8(['double' 0]), timestep=0}
      mask prompts: model "Data Model:"; path "Data Model Path:"; myType "Data Type:"; timestep "MATLAB timestep:"
      mask help:
      | This block reads a scalar value from the pb file.
      |
      | The supported data types are:
      | - double
      | - single
      | - uint32
      | - int32
      mask Display: fprintf('sfun')
  Speed : Outport
  wires:
  sfun/1 -> BusSelector/1
  BusSelector/1 -> Speed/1  "<value>"

== system acc_mpc/Roewe_550_S_Sedan_1/State2PathFollowerCnv ==
  State BUS : Inport  OutDataTypeStr=Bus: PRESCAN_STATEACTUATORDATA
  Bus Selector : BusSelector  OutputSignals=AngularVelocityYaw,VelocityX,VelocityY,PositionX,PositionY,OrientationYaw
  Radians to Degrees : simulink_extras/Transformations/Radians to Degrees
  Radians to Degrees1 : simulink_extras/Transformations/Radians to Degrees
  SELF2PathFollowerMux : Mux  Tag=SELF2PathFollowerMux  Inputs=3
  velocity magnitude : Math  Operator=hypot  SignedPower=on  SaturateOnIntegerOverflow=on
  Yaw rate [deg/s] : Outport  VectorParamsAs1DForOutWhenUnconnected=off
  velocity [m/s] : Outport  Port=2  VectorParamsAs1DForOutWhenUnconnected=off
  position x,y,Y [m,m,deg] : Outport  Port=3  VectorParamsAs1DForOutWhenUnconnected=off
  wires:
  Radians to Degrees1/1 -> Yaw rate [deg/s]/1
  Bus Selector/1 -> Radians to Degrees1/1  "<AngularVelocityYaw>"
  velocity magnitude/1 -> velocity [m/s]/1
  SELF2PathFollowerMux/1 -> position x,y,Y [m,m,deg]/1
  State BUS/1 -> Bus Selector/1
  Bus Selector/2 -> velocity magnitude/1  "<VelocityX>"
  Bus Selector/3 -> velocity magnitude/2  "<VelocityY>"
  Radians to Degrees/1 -> SELF2PathFollowerMux/3
  Bus Selector/6 -> Radians to Degrees/1  "<OrientationYaw>"
  Bus Selector/4 -> SELF2PathFollowerMux/1  "<PositionX>"
  Bus Selector/5 -> SELF2PathFollowerMux/2  "<PositionY>"

== system acc_mpc/Audi_A3_1/AIR_1_Demux/Activate_Switch ==
  BeamID : Inport
  Heading : Inport  Port=2
  Constant : Constant  Value=0
  Product1 : Product  RndMeth=Zero
  Relational Operator : RelationalOperator  Operator=~=  OutDataTypeStr=boolean  RndMeth=Nearest
  On/Off : Outport  VectorParamsAs1DForOutWhenUnconnected=off
  wires:
  Heading/1 -> Product1/2
  Product1/1 -> On/Off/1
  BeamID/1 -> Relational Operator/2
  Relational Operator/1 -> Product1/1
  Constant/1 -> Relational Operator/1

== system acc_mpc/Audi_A3_1/AIR_1_Demux/Signal2ArrayOfSignals1 ==
  note: Initial state of Previous vector block
      | set to zeros(VECTORLENGTH,1)
  note: Set mask parameter VECTORLENGTH
      |  to MAXMESSAGES
  LoopIndex : Inport
  Element : Inport  Port=2
  Assignment : Assignment  IndexOptions=Index vector (port)  Indices=1  OutputSizes=1
  Previous vector : Memory  InitialCondition=zeros(VECTORLENGTH,1)  InheritSampleTime=on
  ArrayofElements : Outport  VectorParamsAs1DForOutWhenUnconnected=off
  wires:
  Assignment/1 -> Previous vector/1, ArrayofElements/1
  Previous vector/1 -> Assignment/1
  LoopIndex/1 -> Assignment/3
  Element/1 -> Assignment/2

== system acc_mpc/Audi_A3_1/AIR_1_Demux/Signal2ArrayOfSignals2 ==
  note: Initial state of Previous vector block
      | set to zeros(VECTORLENGTH,1)
  note: Set mask parameter VECTORLENGTH
      |  to MAXMESSAGES
  LoopIndex : Inport
  Element : Inport  Port=2
  Assignment : Assignment  IndexOptions=Index vector (port)  Indices=1  OutputSizes=1
  Previous vector : Memory  InitialCondition=zeros(VECTORLENGTH,1)  InheritSampleTime=on
  ArrayofElements : Outport  VectorParamsAs1DForOutWhenUnconnected=off
  wires:
  Assignment/1 -> Previous vector/1, ArrayofElements/1
  Previous vector/1 -> Assignment/1
  LoopIndex/1 -> Assignment/3
  Element/1 -> Assignment/2

== system acc_mpc/Audi_A3_1/AIR_1_Demux/Signal2ArrayOfSignals3 ==
  note: Initial state of Previous vector block
      | set to zeros(VECTORLENGTH,1)
  note: Set mask parameter VECTORLENGTH
      |  to MAXMESSAGES
  LoopIndex : Inport
  Element : Inport  Port=2
  Assignment : Assignment  IndexOptions=Index vector (port)  Indices=1  OutputSizes=1
  Previous vector : Memory  InitialCondition=zeros(VECTORLENGTH,1)  InheritSampleTime=on
  ArrayofElements : Outport  VectorParamsAs1DForOutWhenUnconnected=off
  wires:
  Assignment/1 -> Previous vector/1, ArrayofElements/1
  Previous vector/1 -> Assignment/1
  LoopIndex/1 -> Assignment/3
  Element/1 -> Assignment/2

== system acc_mpc/Audi_A3_1/AIR_1_Demux/Signal2ArrayOfSignals4 ==
  note: Initial state of Previous vector block
      | set to zeros(VECTORLENGTH,1)
  note: Set mask parameter VECTORLENGTH
      |  to MAXMESSAGES
  LoopIndex : Inport
  Element : Inport  Port=2
  Assignment : Assignment  IndexOptions=Index vector (port)  Indices=1  OutputSizes=1
  Previous vector : Memory  InitialCondition=zeros(VECTORLENGTH,1)  InheritSampleTime=on
  ArrayofElements : Outport  VectorParamsAs1DForOutWhenUnconnected=off
  wires:
  Assignment/1 -> Previous vector/1, ArrayofElements/1
  Previous vector/1 -> Assignment/1
  LoopIndex/1 -> Assignment/3
  Element/1 -> Assignment/2

== system acc_mpc/Audi_A3_1/AIR_1_Demux/Signal2ArrayOfSignals5 ==
  note: Initial state of Previous vector block
      | set to zeros(VECTORLENGTH,1)
  note: Set mask parameter VECTORLENGTH
      |  to MAXMESSAGES
  LoopIndex : Inport
  Element : Inport  Port=2
  Assignment : Assignment  IndexOptions=Index vector (port)  Indices=1  OutputSizes=1
  Previous vector : Memory  InitialCondition=zeros(VECTORLENGTH,1)  InheritSampleTime=on
  ArrayofElements : Outport  VectorParamsAs1DForOutWhenUnconnected=off
  wires:
  Assignment/1 -> Previous vector/1, ArrayofElements/1
  Previous vector/1 -> Assignment/1
  LoopIndex/1 -> Assignment/3
  Element/1 -> Assignment/2

== system acc_mpc/Audi_A3_1/AIR_1_Demux/Signal2ArrayOfSignals6 ==
  note: Initial state of Previous vector block
      | set to zeros(VECTORLENGTH,1)
  note: Set mask parameter VECTORLENGTH
      |  to MAXMESSAGES
  LoopIndex : Inport
  Element : Inport  Port=2
  Assignment : Assignment  IndexOptions=Index vector (port)  Indices=1  OutputSizes=1
  Previous vector : Memory  InitialCondition=zeros(VECTORLENGTH,1)  InheritSampleTime=on
  ArrayofElements : Outport  VectorParamsAs1DForOutWhenUnconnected=off
  wires:
  Assignment/1 -> Previous vector/1, ArrayofElements/1
  Previous vector/1 -> Assignment/1
  LoopIndex/1 -> Assignment/3
  Element/1 -> Assignment/2

== system acc_mpc/Audi_A3_1/AIR_1_Demux/Signal2ArrayOfSignals7 ==
  note: Initial state of Previous vector block
      | set to zeros(VECTORLENGTH,1)
  note: Set mask parameter VECTORLENGTH
      |  to MAXMESSAGES
  LoopIndex : Inport
  Element : Inport  Port=2
  Assignment : Assignment  IndexOptions=Index vector (port)  Indices=1  OutputSizes=1
  Previous vector : Memory  InitialCondition=zeros(VECTORLENGTH,1)  InheritSampleTime=on
  ArrayofElements : Outport  VectorParamsAs1DForOutWhenUnconnected=off
  wires:
  Assignment/1 -> Previous vector/1, ArrayofElements/1
  Previous vector/1 -> Assignment/1
  LoopIndex/1 -> Assignment/3
  Element/1 -> Assignment/2

== system acc_mpc/Audi_A3_1/AIR_3_Demux/Activate_Switch ==
  BeamID : Inport
  Heading : Inport  Port=2
  Constant : Constant  Value=0
  Product1 : Product  RndMeth=Zero
  Relational Operator : RelationalOperator  Operator=~=  OutDataTypeStr=boolean  RndMeth=Nearest
  On/Off : Outport  VectorParamsAs1DForOutWhenUnconnected=off
  wires:
  Heading/1 -> Product1/2
  Product1/1 -> On/Off/1
  BeamID/1 -> Relational Operator/2
  Relational Operator/1 -> Product1/1
  Constant/1 -> Relational Operator/1

== system acc_mpc/Audi_A3_1/AIR_3_Demux/Signal2ArrayOfSignals1 ==
  note: Initial state of Previous vector block
      | set to zeros(VECTORLENGTH,1)
  note: Set mask parameter VECTORLENGTH
      |  to MAXMESSAGES
  LoopIndex : Inport
  Element : Inport  Port=2
  Assignment : Assignment  IndexOptions=Index vector (port)  Indices=1  OutputSizes=1
  Previous vector : Memory  InitialCondition=zeros(VECTORLENGTH,1)  InheritSampleTime=on
  ArrayofElements : Outport  VectorParamsAs1DForOutWhenUnconnected=off
  wires:
  Assignment/1 -> Previous vector/1, ArrayofElements/1
  Previous vector/1 -> Assignment/1
  LoopIndex/1 -> Assignment/3
  Element/1 -> Assignment/2

== system acc_mpc/Audi_A3_1/AIR_3_Demux/Signal2ArrayOfSignals2 ==
  note: Initial state of Previous vector block
      | set to zeros(VECTORLENGTH,1)
  note: Set mask parameter VECTORLENGTH
      |  to MAXMESSAGES
  LoopIndex : Inport
  Element : Inport  Port=2
  Assignment : Assignment  IndexOptions=Index vector (port)  Indices=1  OutputSizes=1
  Previous vector : Memory  InitialCondition=zeros(VECTORLENGTH,1)  InheritSampleTime=on
  ArrayofElements : Outport  VectorParamsAs1DForOutWhenUnconnected=off
  wires:
  Assignment/1 -> Previous vector/1, ArrayofElements/1
  Previous vector/1 -> Assignment/1
  LoopIndex/1 -> Assignment/3
  Element/1 -> Assignment/2

== system acc_mpc/Audi_A3_1/AIR_3_Demux/Signal2ArrayOfSignals3 ==
  note: Initial state of Previous vector block
      | set to zeros(VECTORLENGTH,1)
  note: Set mask parameter VECTORLENGTH
      |  to MAXMESSAGES
  LoopIndex : Inport
  Element : Inport  Port=2
  Assignment : Assignment  IndexOptions=Index vector (port)  Indices=1  OutputSizes=1
  Previous vector : Memory  InitialCondition=zeros(VECTORLENGTH,1)  InheritSampleTime=on
  ArrayofElements : Outport  VectorParamsAs1DForOutWhenUnconnected=off
  wires:
  Assignment/1 -> Previous vector/1, ArrayofElements/1
  Previous vector/1 -> Assignment/1
  LoopIndex/1 -> Assignment/3
  Element/1 -> Assignment/2

== system acc_mpc/Audi_A3_1/AIR_3_Demux/Signal2ArrayOfSignals4 ==
  note: Initial state of Previous vector block
      | set to zeros(VECTORLENGTH,1)
  note: Set mask parameter VECTORLENGTH
      |  to MAXMESSAGES
  LoopIndex : Inport
  Element : Inport  Port=2
  Assignment : Assignment  IndexOptions=Index vector (port)  Indices=1  OutputSizes=1
  Previous vector : Memory  InitialCondition=zeros(VECTORLENGTH,1)  InheritSampleTime=on
  ArrayofElements : Outport  VectorParamsAs1DForOutWhenUnconnected=off
  wires:
  Assignment/1 -> Previous vector/1, ArrayofElements/1
  Previous vector/1 -> Assignment/1
  LoopIndex/1 -> Assignment/3
  Element/1 -> Assignment/2

== system acc_mpc/Audi_A3_1/AIR_3_Demux/Signal2ArrayOfSignals5 ==
  note: Initial state of Previous vector block
      | set to zeros(VECTORLENGTH,1)
  note: Set mask parameter VECTORLENGTH
      |  to MAXMESSAGES
  LoopIndex : Inport
  Element : Inport  Port=2
  Assignment : Assignment  IndexOptions=Index vector (port)  Indices=1  OutputSizes=1
  Previous vector : Memory  InitialCondition=zeros(VECTORLENGTH,1)  InheritSampleTime=on
  ArrayofElements : Outport  VectorParamsAs1DForOutWhenUnconnected=off
  wires:
  Assignment/1 -> Previous vector/1, ArrayofElements/1
  Previous vector/1 -> Assignment/1
  LoopIndex/1 -> Assignment/3
  Element/1 -> Assignment/2

== system acc_mpc/Audi_A3_1/AIR_3_Demux/Signal2ArrayOfSignals6 ==
  note: Initial state of Previous vector block
      | set to zeros(VECTORLENGTH,1)
  note: Set mask parameter VECTORLENGTH
      |  to MAXMESSAGES
  LoopIndex : Inport
  Element : Inport  Port=2
  Assignment : Assignment  IndexOptions=Index vector (port)  Indices=1  OutputSizes=1
  Previous vector : Memory  InitialCondition=zeros(VECTORLENGTH,1)  InheritSampleTime=on
  ArrayofElements : Outport  VectorParamsAs1DForOutWhenUnconnected=off
  wires:
  Assignment/1 -> Previous vector/1, ArrayofElements/1
  Previous vector/1 -> Assignment/1
  LoopIndex/1 -> Assignment/3
  Element/1 -> Assignment/2

== system acc_mpc/Audi_A3_1/AIR_3_Demux/Signal2ArrayOfSignals7 ==
  note: Initial state of Previous vector block
      | set to zeros(VECTORLENGTH,1)
  note: Set mask parameter VECTORLENGTH
      |  to MAXMESSAGES
  LoopIndex : Inport
  Element : Inport  Port=2
  Assignment : Assignment  IndexOptions=Index vector (port)  Indices=1  OutputSizes=1
  Previous vector : Memory  InitialCondition=zeros(VECTORLENGTH,1)  InheritSampleTime=on
  ArrayofElements : Outport  VectorParamsAs1DForOutWhenUnconnected=off
  wires:
  Assignment/1 -> Previous vector/1, ArrayofElements/1
  Previous vector/1 -> Assignment/1
  LoopIndex/1 -> Assignment/3
  Element/1 -> Assignment/2
